simulink model "task5"  (R2024b)
settings: Solver=VariableStepAuto  StartTime=0.0  StopTime=10.0  RelTol=1e-3
settings Model: Creator=33657  LastModifiedBy=33657

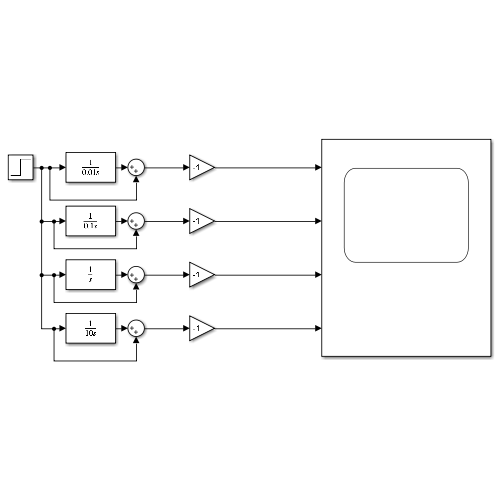
[thumbnail: Simulink's stored preview of the top-level diagram]
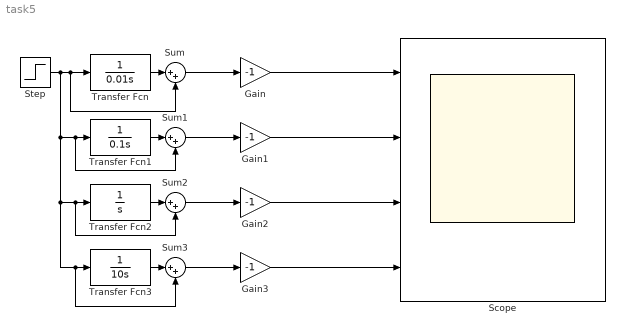
== system task5 ==
  Gain{,1..3} (4 alike) : Gain  Gain=-1
  Scope : Scope  NumInputPorts=4
  Step : Step  SampleTime=0
  Sum{,1..3} (4 alike) : Sum  Inputs=|++
  Transfer Fcn : TransferFcn  Denominator=[0.01 0]
  Transfer Fcn1 : TransferFcn  Denominator=[0.1 0]
  Transfer Fcn2 : TransferFcn  Denominator=[1 0]
  Transfer Fcn3 : TransferFcn  Denominator=[10 0]
  wires:
  Sum/1 -> Gain/1
  Gain/1 -> Scope/1
  Step/1 -> Sum3/2, Transfer Fcn3/1, Sum2/2, Transfer Fcn2/1, Sum1/2, Transfer Fcn1/1, Transfer Fcn/1, Sum/2
  Sum1/1 -> Gain1/1
  Sum2/1 -> Gain2/1
  Sum3/1 -> Gain3/1
  Gain1/1 -> Scope/2
  Gain2/1 -> Scope/3
  Gain3/1 -> Scope/4
  Transfer Fcn/1 -> Sum/1
  Transfer Fcn1/1 -> Sum1/1
  Transfer Fcn2/1 -> Sum2/1
  Transfer Fcn3/1 -> Sum3/1
